simulink model "MotorFOCShared"  (R2024b)
settings: Solver=FixedStepDiscrete  StartTime=0.0  StopTime=6  FixedStep=1e-4  RelTol=1e-3
values from neighbouring files (symbols this model uses):
  CurrKi = 35.0    [motor_comparison.sldd]
  CurrKp = 0.26    [motor_comparison.sldd]
  flux = 0.016884    [motor_comparison.sldd]
  Pn = 2.0    [motor_comparison.sldd]
  spd_ki = 0.00144    [motor_comparison.sldd]
  spd_kp = 0.003389    [motor_comparison.sldd]
  Udc = 24.0    [motor_comparison.sldd]
undefined symbols (not defined in the file or in its folder): curr_d_ki, curr_d_kp, curr_q_ki, curr_q_kp, DiscIntNeverNeededParam
libraries: slpidlib x3, mcbplantlib x1, simulink x1, autolibpmsmexterior x1
settings Model: DataDictionary=motor_comparison.sldd  Creator=Administrator  LastModifiedBy=lxy
settings OptimizationCC: DefaultParameterBehavior=Inlined  UseDivisionForNetSlopeComputation=on  GainParamInheritBuiltInType=on  UseFloatMulNetSlope=on  InlineInvariantSignals=on  PassReuseOutputArgsAs=Individual arguments  ZeroExternalMemoryAtStartup=off  ZeroInternalMemoryAtStartup=off  NoFixptDivByZeroProtection=on  EfficientFloat2IntCast=on  LifeSpan=1  OptimizeBlockOrder=speed  DifferentSizesBufferReuse=on  EfficientTunableParamExpr=on
settings DebuggingCC: ParameterPrecisionLossMsg=none  ParameterTunabilityLossMsg=error  UnconnectedInputMsg=warning  UnconnectedOutputMsg=warning  UnconnectedLineMsg=warning
settings HardwareCC: ProdBitPerPointer=32  ProdBitPerSizeT=32  ProdBitPerPtrDiffT=32  ProdLargestAtomicInteger=Long  ProdLargestAtomicFloat=Double  ProdWordSize=32  ProdLongLongMode=on  ProdHWDeviceType=ARM Compatible->ARM Cortex-M
settings ModelReferenceCC: EnableRefExpFcnMdlSchedulingChecks=on  ModelReferenceNumInstancesAllowed=Single
settings SFSimCC: MATLABDynamicMemAlloc=off
settings RTWCC: Description=Embedded Coder  SystemTargetFile=ert.tlc  GenCodeOnly=on  TemplateMakefile=ert_default_tmf  GenerateReport=on  LaunchReport=on  GenerateCodeReplacementReport=on  GPUComputeCapability=3.5  DLArmComputeVersion=19.05
settings CodeAppCC: ForceParamTrailComments=on  IgnoreCustomStorageClasses=off  OperatorAnnotations=on  SimulinkDataObjDesc=on  SFDataObjDesc=on  CustomSymbolStrGlobalVar=rt$N$M  CustomSymbolStrType=$N$M  CustomSymbolStrFcn=$N$M$F  CustomSymbolStrMacro=$N$M  InsertBlockDesc=on
settings ERTTargetCC: TargetLangStandard=C99 (ISO)  GenerateSampleERTMain=on  IncludeMdlTerminateFcn=off  CombineSignalStateStructs=on  SupportComplex=off  SupportNonInlinedSFcns=on  ERTCustomFileTemplate=example_file_process.tlc  ERTFilePackagingFormat=CompactWithDataFile  DynamicArrayContainerType=coder::array

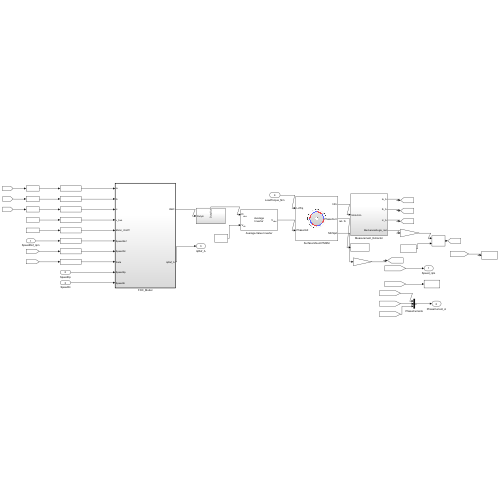
[thumbnail: Simulink's stored preview of the top-level diagram]
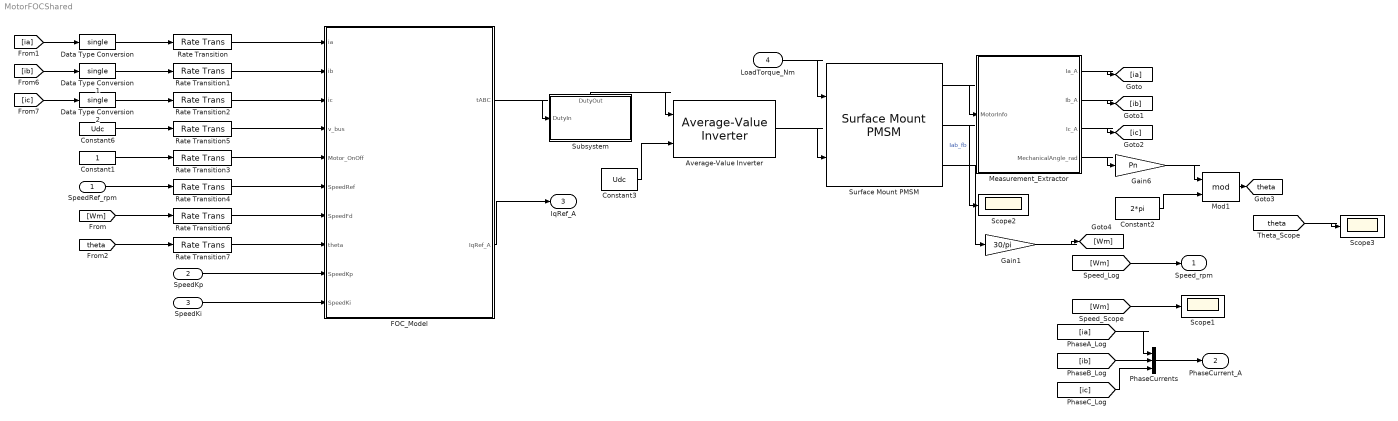
== system MotorFOCShared ==
  SpeedRef_rpm : Inport  OutDataTypeStr=single  SampleTime=1e-4
  SpeedKp : Inport  Port=2  OutDataTypeStr=single  SampleTime=1e-4
  SpeedKi : Inport  Port=3  OutDataTypeStr=single  SampleTime=1e-4
  LoadTorque_Nm : Inport  Port=4  OutDataTypeStr=double  SampleTime=1e-4
  Average-Value Inverter : mcbplantlib/Average-Value Inverter
  Constant1 : Constant  OutDataTypeStr=single
  Constant2 : Constant  Value=2*pi  OutDataTypeStr=single
  Constant3 : Constant  Value=Udc
  Constant6 : Constant  Value=Udc  OutDataTypeStr=single
  Data Type Conversion : DataTypeConversion  OutDataTypeStr=single  SaturateOnIntegerOverflow=off  RndMeth=Floor
  Data Type Conversion1 : DataTypeConversion  OutDataTypeStr=single  SaturateOnIntegerOverflow=off  RndMeth=Floor
  Data Type Conversion2 : DataTypeConversion  OutDataTypeStr=single  SaturateOnIntegerOverflow=off  RndMeth=Floor
  FOC_Model : Subsystem  TreatAsAtomicUnit=on
  Gain1 : Gain  Gain=30/pi  OutDataTypeStr=single
  Gain6 : Gain  Gain=Pn  OutDataTypeStr=single
  Measurement_Extractor : Subsystem
  Mod1 : Math  Operator=mod  OutputSignalType=real
  PhaseCurrents : Mux  Inputs=3
  Rate Transition{,1..7} (8 alike) : RateTransition
  Scope1 : Scope
  Scope2 : Scope
  Scope3 : Scope
  Subsystem : Subsystem
      settings: PortSchema="{\"entries\":[{\"content\":{\"sides\":[{\"content\":{\"connectorIds\":[\"In1\"]},\"type\":\"ConnectorPlacement.EquallySpacedRectSide\",\"uuid\":\"8ccc51de-fa2a-4900-80a3-4cdf9aa76f01\"},{\"content\":{\"connectorIds\":[],\"side\":\"RIGHT\"},\"type\":\"ConnectorPlacement.EquallySpacedRectSide\",\"uuid\":\"32c06e0d-3f1d-4948-af96-e310e54308a0\"},{\"content\":{\"connectorIds\":[\"Out1\"],\"side\":\"TOP\"},\"type\":\"ConnectorPlacement.EquallySpacedRectSide\",\"uuid\":\"a9066067-2c54-42a8-b4d7-fb86ac71b860\"}]},\"type\":\"ConnectorPlacement.EquallySpacedConnector\",\"uuid\":\"e4576975-acad-4e16-822f-2c2e7f23d7a7\"}],\"packageUris\":[\"http://schema.mathworks.com/mf0/Connector/R2020b\"],\"version\":\"1.0\"}"
  Surface Mount PMSM : autolibpmsmexterior/Surface Mount PMSM  port_config=Torque  sim_type=Discrete  Ts=1e-4  P=Pn  Rs=Rs  Ldq_=L  KConstText=Permanent flux linkage constant (lambda_pm):  lambda_pm=flux  Ke=0.0059268  Kt=0.061  mechanical=[75e-6, 8e-5, 0]  idq0=[0 0]  theta_init=4/5  omega_init=0  KConst=flux  lambda_pm_calc=flux  RefBlkName='autolibpmsmexterior/Surface Mount PMSM'  aMode=5  Ldq="[0.0017      0.0017]"
  Speed_rpm : Outport
  PhaseCurrent_A : Outport  Port=2
  IqRef_A : Outport  Port=3
  tag scope: theta=global
  wires:
  Constant3/1 -> Average-Value Inverter/2
  Subsystem/1(DutyOut) -> Average-Value Inverter/1
  Average-Value Inverter/1 -> Surface Mount PMSM/2
  Surface Mount PMSM/3 -> Gain1/1
  [ia] -> Data Type Conversion/1
  [ic] -> Data Type Conversion2/1
  [ib] -> Data Type Conversion1/1
  Data Type Conversion/1 -> Rate Transition/1
  Data Type Conversion1/1 -> Rate Transition1/1
  Data Type Conversion2/1 -> Rate Transition2/1
  Constant6/1 -> Rate Transition5/1
  Surface Mount PMSM/2 -> Scope2/1  "Iab_fb"
  Gain6/1 -> Mod1/1
  Constant2/1 -> Mod1/2
  Mod1/1 -> [theta]
  Constant1/1 -> Rate Transition3/1
  Gain1/1 -> [Wm]
  Rate Transition/1 -> FOC_Model/1(ia)
  Rate Transition1/1 -> FOC_Model/2(ib)
  Rate Transition2/1 -> FOC_Model/3(ic)
  Rate Transition5/1 -> FOC_Model/4(v_bus)
  Rate Transition3/1 -> FOC_Model/5(Motor_OnOff)
  FOC_Model/1(tABC) -> Subsystem/1(DutyIn)
  Rate Transition4/1 -> FOC_Model/6(SpeedRef)
  Rate Transition6/1 -> FOC_Model/7(SpeedFd)
  Rate Transition7/1 -> FOC_Model/8(theta)
  [theta] -> Rate Transition7/1
  [Wm] -> Rate Transition6/1
  SpeedRef_rpm/1 -> Rate Transition4/1
  LoadTorque_Nm/1 -> Surface Mount PMSM/1
  PhaseCurrents/1 -> PhaseCurrent_A/1
  SpeedKp/1 -> FOC_Model/9(SpeedKp)
  SpeedKi/1 -> FOC_Model/10(SpeedKi)
  FOC_Model/2(IqRef_A) -> IqRef_A/1
  [ia] -> PhaseCurrents/1
  [ib] -> PhaseCurrents/2
  [ic] -> PhaseCurrents/3
  [Wm] -> Speed_rpm/1
  [Wm] -> Scope1/1
  [theta] -> Scope3/1
  Surface Mount PMSM/1 -> Measurement_Extractor/1(MotorInfo)
  Measurement_Extractor/1(Ia_A) -> [ia]
  Measurement_Extractor/2(Ib_A) -> [ib]
  Measurement_Extractor/3(Ic_A) -> [ic]
  Measurement_Extractor/4(MechanicalAngle_rad) -> Gain6/1

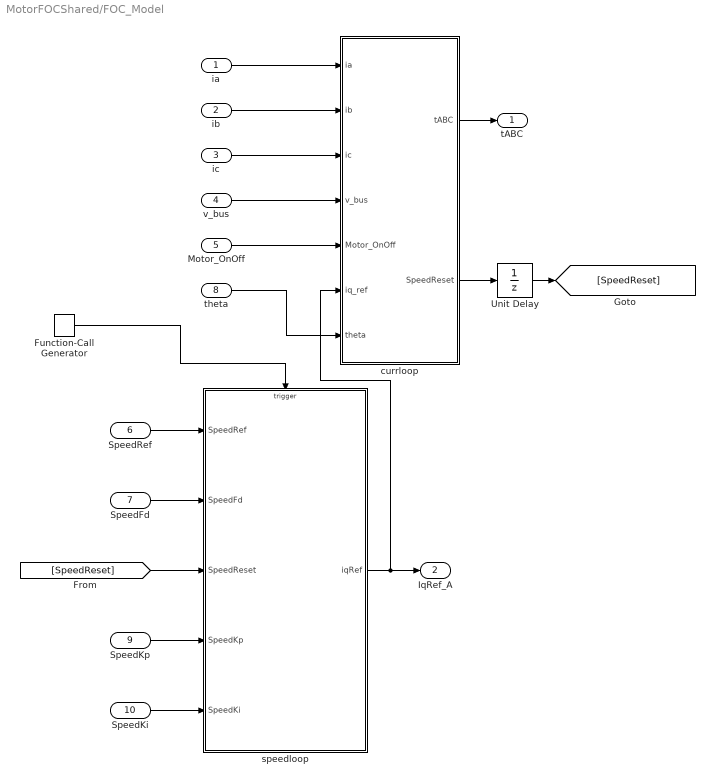
== system MotorFOCShared/FOC_Model ==
  ia : Inport
  ib : Inport  Port=2
  ic : Inport  Port=3
  v_bus : Inport  Port=4
  Motor_OnOff : Inport  Port=5
  SpeedRef : Inport  Port=6
  SpeedFd : Inport  Port=7
  theta : Inport  Port=8
  SpeedKp : Inport  Port=9  OutDataTypeStr=single
  SpeedKi : Inport  Port=10  OutDataTypeStr=single
  Function-Call Generator : simulink/Ports & Subsystems/Function-Call Generator  sample_time=1e-3  numberOfIterations=1  DisallowWideOutput=off
  Unit Delay : UnitDelay  SampleTime=-1  HasFrameUpgradeWarning=on
  currloop : Subsystem  TreatAsAtomicUnit=on
  speedloop : Subsystem
  tABC : Outport
  IqRef_A : Outport  Port=2
  wires:
  SpeedKi/1 -> speedloop/5(SpeedKi)
  SpeedKp/1 -> speedloop/4(SpeedKp)
  currloop/1(tABC) -> tABC/1
  [SpeedReset] -> speedloop/3(SpeedReset)
  theta/1 -> currloop/7(theta)
  Function-Call Generator/1 -> speedloop/Trigger
  SpeedRef/1 -> speedloop/1(SpeedRef)
  ib/1 -> currloop/2(ib)
  Motor_OnOff/1 -> currloop/5(Motor_OnOff)
  ia/1 -> currloop/1(ia)
  ic/1 -> currloop/3(ic)
  SpeedFd/1 -> speedloop/2(SpeedFd)
  v_bus/1 -> currloop/4(v_bus)
  speedloop/1(iqRef) -> IqRef_A/1, currloop/6(iq_ref)
  currloop/2(SpeedReset) -> Unit Delay/1
  Unit Delay/1 -> [SpeedReset]

== system MotorFOCShared/Measurement_Extractor ==
  MotorInfo : Inport
  Phase_And_Position : BusSelector  OutputSignals=IaStator,IbStator,IcStator,MtrPos
  Ia_A : Outport
  Ib_A : Outport  Port=2
  Ic_A : Outport  Port=3
  MechanicalAngle_rad : Outport  Port=4
  wires:
  Phase_And_Position/4 -> MechanicalAngle_rad/1  "<MtrPos>"
  Phase_And_Position/2 -> Ib_A/1  "<IbStator>"
  MotorInfo/1 -> Phase_And_Position/1
  Phase_And_Position/3 -> Ic_A/1  "<IcStator>"
  Phase_And_Position/1 -> Ia_A/1  "<IaStator>"

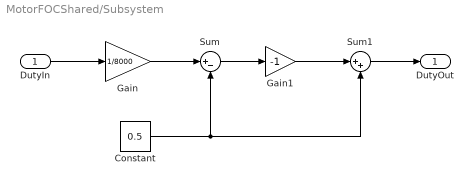
== system MotorFOCShared/Subsystem ==
  DutyIn : Inport
  Constant : Constant  Value=0.5  SampleTime=-1
  Gain : Gain  Gain=1/8000  ParamDataTypeStr=single
  Gain1 : Gain  Gain=-1
  Sum : Sum  Inputs=|+-
  Sum1 : Sum  Inputs=|++
  DutyOut : Outport
  wires:
  Sum/1 -> Gain1/1
  Constant/1 -> Sum1/2, Sum/2
  DutyIn/1 -> Gain/1
  Gain1/1 -> Sum1/1
  Sum1/1 -> DutyOut/1
  Gain/1 -> Sum/1

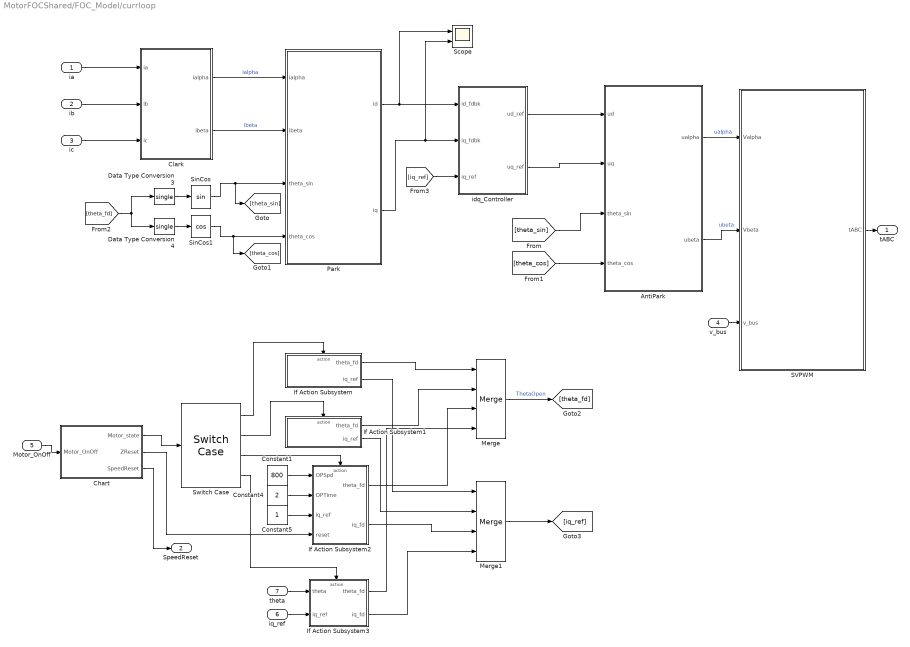
== system MotorFOCShared/FOC_Model/currloop ==
  ia : Inport
  ib : Inport  Port=2
  ic : Inport  Port=3
  v_bus : Inport  Port=4
  Motor_OnOff : Inport  Port=5
  iq_ref : Inport  Port=6
  theta : Inport  Port=7
  AntiPark : Subsystem
  Chart : Stateflow chart  TreatAsAtomicUnit=on
  Clark : Subsystem
  Constant1 : Constant  Value=800  OutDataTypeStr=single
  Constant4 : Constant  Value=2  OutDataTypeStr=single
  Constant5 : Constant  OutDataTypeStr=single
  Data Type Conversion3 : DataTypeConversion  OutDataTypeStr=single  SaturateOnIntegerOverflow=off  RndMeth=Floor
  Data Type Conversion4 : DataTypeConversion  OutDataTypeStr=single  SaturateOnIntegerOverflow=off  RndMeth=Floor
  If Action Subsystem : Subsystem  TreatAsAtomicUnit=on
  If Action Subsystem1 : Subsystem  TreatAsAtomicUnit=on
  If Action Subsystem2 : Subsystem  TreatAsAtomicUnit=on
  If Action Subsystem3 : Subsystem  TreatAsAtomicUnit=on
  Merge : Merge  Inputs=4
  Merge1 : Merge  Inputs=4
  Park : Subsystem
  SVPWM : Subsystem  TreatAsAtomicUnit=on
  Scope : Scope  NumInputPorts=2
  SinCos : Trigonometry
  SinCos1 : Trigonometry  Operator=cos
  Switch Case : SwitchCase  CaseConditions={1,2,3,4}  ShowDefaultCase=off
  idq_Controller : Subsystem
  tABC : Outport
  SpeedReset : Outport  Port=2
  wires:
  Data Type Conversion4/1 -> SinCos1/1
  Data Type Conversion3/1 -> SinCos/1
  AntiPark/2(ubeta) -> SVPWM/2(Vbeta)  "ubeta"
  AntiPark/1(ualpha) -> SVPWM/1(Valpha)  "ualpha"
  [theta_cos] -> AntiPark/4(theta_cos)
  [theta_sin] -> AntiPark/3(theta_sin)
  SinCos/1 -> Park/3(theta_sin), [theta_sin]
  [theta_fd] -> Data Type Conversion3/1, Data Type Conversion4/1
  SinCos1/1 -> Park/4(theta_cos), [theta_cos]
  v_bus/1 -> SVPWM/3(v_bus)
  SVPWM/1(tABC) -> tABC/1
  ib/1 -> Clark/2(ib)
  ia/1 -> Clark/1(ia)
  ic/1 -> Clark/3(ic)
  Clark/1(ialpha) -> Park/1(ialpha)  "ialpha"
  Clark/2(ibeta) -> Park/2(ibeta)  "ibeta"
  idq_Controller/1(ud_ref) -> AntiPark/1(ud)
  idq_Controller/2(uq_ref) -> AntiPark/2(uq)
  Park/1(id) -> Scope/1, idq_Controller/1(id_fdbk)
  Park/2(iq) -> Scope/2, idq_Controller/2(iq_fdbk)
  [iq_ref] -> idq_Controller/3(iq_ref)
  Constant1/1 -> If Action Subsystem2/1(OPSpd)
  iq_ref/1 -> If Action Subsystem3/2(iq_ref)
  Switch Case/2 -> If Action Subsystem1/Action
  Chart/1(Motor_state) -> Switch Case/1
  theta/1 -> If Action Subsystem3/1(theta)
  Switch Case/4 -> If Action Subsystem3/Action
  Constant4/1 -> If Action Subsystem2/2(OPTime)
  Constant5/1 -> If Action Subsystem2/3(iq_ref)
  Switch Case/1 -> If Action Subsystem/Action
  Switch Case/3 -> If Action Subsystem2/Action
  If Action Subsystem/1(theta_fd) -> Merge/1
  If Action Subsystem1/1(theta_fd) -> Merge/2
  If Action Subsystem2/1(theta_fd) -> Merge/3
  If Action Subsystem3/1(theta_fd) -> Merge/4
  If Action Subsystem/2(iq_ref) -> Merge1/1
  If Action Subsystem1/2(iq_ref) -> Merge1/2
  If Action Subsystem2/2(iq_fd) -> Merge1/3
  If Action Subsystem3/2(iq_fd) -> Merge1/4
  Merge/1 -> [theta_fd]  "ThetaOpen"
  Merge1/1 -> [iq_ref]
  Motor_OnOff/1 -> Chart/1(Motor_OnOff)
  Chart/2(ZReset) -> If Action Subsystem2/4(reset)
  Chart/3(SpeedReset) -> SpeedReset/1

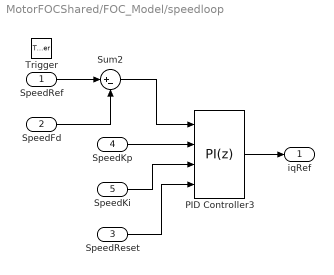
== system MotorFOCShared/FOC_Model/speedloop ==
  SpeedRef : Inport
  SpeedFd : Inport  Port=2
  SpeedReset : Inport  Port=3
  SpeedKp : Inport  Port=4  OutDataTypeStr=single
  SpeedKi : Inport  Port=5  OutDataTypeStr=single
  Trigger : TriggerPort  TriggerType=function-call  VariantControl=(inherit)  PortDimensions=1
  PID Controller3 : slpidlib/PID Controller  Controller=PI  Form=Parallel  TimeDomain=Discrete-time  UseExternalTs=off  SampleTime=-1  IntegratorMethod=Forward Euler  FilterMethod=Forward Euler  ControllerParametersSource=external  P=spd_kp  I=spd_ki  UseKiTs=off  D=0  UseExternalDerivativeSource=off  N=100  UseFilter=on  TunerSelectOption=Transfer Function Based (PID Tuner App)  InitialConditionSource=internal  InitialConditionForIntegrator=0  InitialConditionForFilter=0  DifferentiatorICPrevScaledInput=0  ExternalReset=rising  TrackingMode=off  Kt=1  LimitOutput=on  SatLimitsSource=internal  UpperSaturationLimit=3  LowerSaturationLimit=-3  LinearizeAsGain=on  AntiWindupMode=clamping  Kb=0.013  LimitIntegrator=off  UpperIntegratorSaturationLimit=inf  LowerIntegratorSaturationLimit=-inf  PGainOutDataTypeStr=single  PProdOutDataTypeStr=single  POutMin=[]  POutMax=[]  IGainOutDataTypeStr=single  IProdOutDataTypeStr=single  IOutMin=[]  IOutMax=[]  DOutMin=[]  DOutMax=[]  NOutMin=[]  NOutMax=[]  SumOutDataTypeStr=single  SumOutMin=[]  SumOutMax=[]  SaturationOutDataTypeStr=single  SaturationOutMin=[]  SaturationOutMax=[]  PParamMin=[]  PParamMax=[]  IParamMin=[]  IParamMax=[]  DParamMin=[]  DParamMax=[]  NParamMin=[]  NParamMax=[]  KbParamMin=[]  KbParamMax=[]  KtParamMin=[]  KtParamMax=[]  KbOutMin=[]  KbOutMax=[]  KtOutMin=[]  KtOutMax=[]  IntegratorOutMin=[]  IntegratorOutMax=[]  FilterOutMin=[]  FilterOutMax=[]  SumI1OutMin=[]  SumI1OutMax=[]  SumI2OutMin=[]  SumI2OutMax=[]  SumI3OutMin=[]  SumI3OutMax=[]  SumI4OutMin=[]  SumI4OutMax=[]  SumDOutMin=[]  SumDOutMax=[]  DifferentiatorOutMin=[]  DifferentiatorOutMax=[]  FilterDiffOutCoefMin=[]  FilterDiffOutCoefMax=[]  ReciprocalOutMin=[]  ReciprocalOutMax=[]  SumDenOutMin=[]  SumDenOutMax=[]  SumNumOutMin=[]  SumNumOutMax=[]  DivideOutMin=[]  DivideOutMax=[]  UdiffTsProdOutMin=[]  UdiffTsProdOutMax=[]  NTsProdOutMin=[]  NTsProdOutMax=[]  UintegralTsProdOutMin=[]  UintegralTsProdOutMax=[]  UngainTsProdOutMin=[]  UngainTsProdOutMax=[]  ClampingZeroOutDataTypeStr=Inherit: Inherit via back propagation  ClampingZeroOutMin=[]  ClampingZeroOutMax=[]  FilterDenConstantOutDataTypeStr=Inherit: Inherit via back propagation  FilterDenConstantOutMin=[]  FilterDenConstantOutMax=[]  PCopyOutDataTypeStr=Inherit: Inherit via back propagation  PCopyOutMin=[]  PCopyOutMax=[]  NCopyOutDataTypeStr=Inherit: Inherit via back propagation  NCopyOutMin=[]  NCopyOutMax=[]  IntegratorContinuousStateAttributes=''  IntegratorStateMustResolveToSignalObject=off  IntegratorRTWStateStorageClass=Auto  FilterContinuousStateAttributes=''  FilterStateMustResolveToSignalObject=off  FilterRTWStateStorageClass=Auto  ParallelPVariant=ExternalParameters  IdealPVariant=Disabled  IVariant=ExternalParameters  DVariant=Disabled  IntegratorVariant=Discrete  SatVariant=Enabled  AWVariant=DiscClampingParallel  PCopyVariant=Disabled  TRVariant=Disabled  FdbkBlocksVariant=Forward  IdealPFdbkVariant=Disabled  SatFdbkVariant=Disabled  DerivativeFilterVariant=Disabled  NVariant=Disabled  NCopyVariant=Disabled_SignalSpec  FilterICVariant=Disabled  IntegratorICVariant=InternalICs  ExternalResetVariant=ExternalReset  TRSumVariant=Passthrough  SumFdbkVariant=Disabled  SumVariant=Sum_PI  TsampFilterVariant=InternalTs  TsampNgainVariant=Passthrough  TsampIntegralVariant=Disabled_SignalSpec  ExternalSaturationOutDataTypeStr=single  DerivativeSourceVariant=Disabled  PreIntVariant=InternalPreInt
  Sum2 : Sum  Inputs=|+-  OutDataTypeStr=single  AccumDataTypeStr=single
  iqRef : Outport
  wires:
  SpeedReset/1 -> PID Controller3/4
  SpeedKi/1 -> PID Controller3/3
  SpeedKp/1 -> PID Controller3/2
  SpeedFd/1 -> Sum2/2
  SpeedRef/1 -> Sum2/1
  PID Controller3/1 -> iqRef/1
  Sum2/1 -> PID Controller3/1

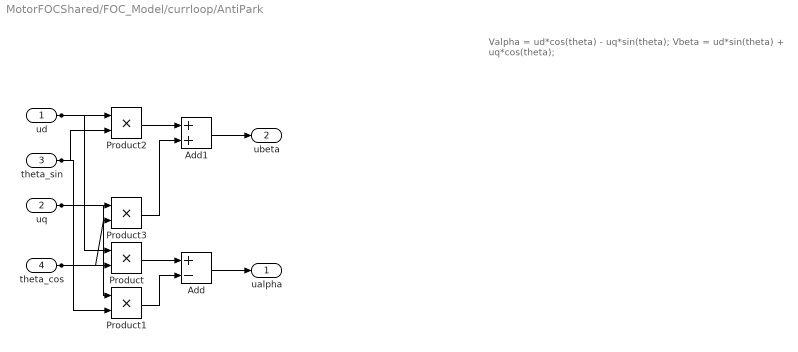
== system MotorFOCShared/FOC_Model/currloop/AntiPark ==
  note: Valpha = ud*cos(theta) - uq*sin(theta);
      | Vbeta = ud*sin(theta) + uq*cos(theta);
  ud : Inport
  uq : Inport  Port=2
  theta_sin : Inport  Port=3
  theta_cos : Inport  Port=4
  Add : Sum  Inputs=+-
  Add1 : Sum
  Product{,1..3} (4 alike) : Product
  ualpha : Outport  OutDataTypeStr=single
  ubeta : Outport  Port=2  OutDataTypeStr=single
  wires:
  ud/1 -> Product/1, Product2/1
  theta_sin/1 -> Product1/2, Product2/2
  Product/1 -> Add/1
  Product2/1 -> Add1/1
  Add/1 -> ualpha/1
  uq/1 -> Product1/1, Product3/1
  Product3/1 -> Add1/2
  theta_cos/1 -> Product3/2, Product/2
  Product1/1 -> Add/2
  Add1/1 -> ubeta/1

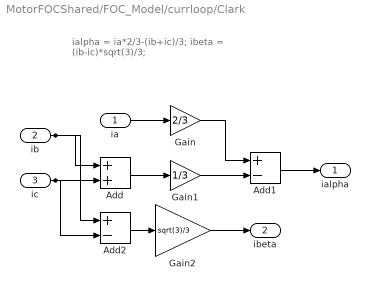
== system MotorFOCShared/FOC_Model/currloop/Clark ==
  note: ialpha = ia*2/3-(ib+ic)/3;
      | ibeta = (ib-ic)*sqrt(3)/3;
  ia : Inport  OutDataTypeStr=single
  ib : Inport  Port=2  OutDataTypeStr=single
  ic : Inport  Port=3  OutDataTypeStr=single
  Add : Sum  OutDataTypeStr=single  AccumDataTypeStr=single
  Add1 : Sum  Inputs=+-  OutDataTypeStr=single  AccumDataTypeStr=single
  Add2 : Sum  Inputs=+-  OutDataTypeStr=single  AccumDataTypeStr=single
  Gain : Gain  Gain=2/3  ParamDataTypeStr=single
  Gain1 : Gain  Gain=1/3  ParamDataTypeStr=single
  Gain2 : Gain  Gain=sqrt(3)/3  ParamDataTypeStr=single
  ialpha : Outport  OutDataTypeStr=single
  ibeta : Outport  Port=2  OutDataTypeStr=single
  wires:
  ib/1 -> Add/1, Add2/1
  Gain/1 -> Add1/1
  ic/1 -> Add/2, Add2/2
  Gain2/1 -> ibeta/1
  Gain1/1 -> Add1/2
  ia/1 -> Gain/1
  Add2/1 -> Gain2/1
  Add/1 -> Gain1/1
  Add1/1 -> ialpha/1

== system MotorFOCShared/FOC_Model/currloop/If Action Subsystem ==
  Action Port : ActionPort  ActionPortLabel=case [ 1 ]:
  Constant : Constant  Value=0  OutDataTypeStr=single
  Constant1 : Constant  Value=0  OutDataTypeStr=single
  theta_fd : Outport
  iq_ref : Outport  Port=2
  wires:
  Constant1/1 -> iq_ref/1
  Constant/1 -> theta_fd/1

== system MotorFOCShared/FOC_Model/currloop/If Action Subsystem1 ==
  Action Port : ActionPort  ActionPortLabel=case [ 2 ]:
  Constant : Constant  Value=0  OutDataTypeStr=single
  Constant1 : Constant  OutDataTypeStr=single
  theta_fd : Outport
  iq_ref : Outport  Port=2
  wires:
  Constant1/1 -> iq_ref/1
  Constant/1 -> theta_fd/1

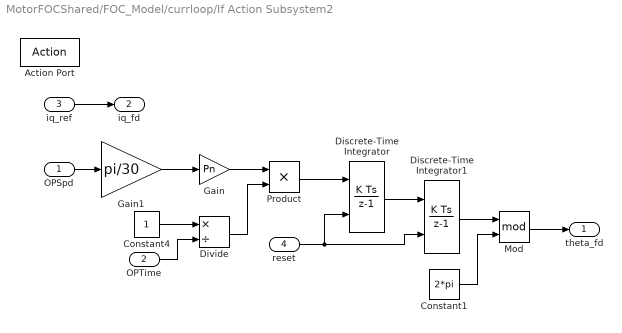
== system MotorFOCShared/FOC_Model/currloop/If Action Subsystem2 ==
  OPSpd : Inport  OutDataTypeStr=single  PortDimensions=1
  OPTime : Inport  Port=2  OutDataTypeStr=single  PortDimensions=1
  iq_ref : Inport  Port=3
  reset : Inport  Port=4
  Action Port : ActionPort  ActionPortLabel=case [ 3 ]:
  Constant1 : Constant  Value=2*pi  OutDataTypeStr=single
  Constant4 : Constant  OutDataTypeStr=single
  Discrete-Time Integrator : DiscreteIntegrator  ExternalReset=rising  SampleTime=-1  ICPrevOutput=DiscIntNeverNeededParam  ICPrevScaledInput=DiscIntNeverNeededParam
  Discrete-Time Integrator1 : DiscreteIntegrator  ExternalReset=rising  SampleTime=-1  ICPrevOutput=DiscIntNeverNeededParam  ICPrevScaledInput=DiscIntNeverNeededParam
  Divide : Product  Inputs=*/  OutDataTypeStr=single
  Gain : Gain  Gain=Pn
  Gain1 : Gain  Gain=pi/30  OutDataTypeStr=single
  Mod : Math  Operator=mod
  Product : Product  OutDataTypeStr=single
  theta_fd : Outport
  iq_fd : Outport  Port=2
  wires:
  Gain/1 -> Product/1
  Discrete-Time Integrator1/1 -> Mod/1
  OPTime/1 -> Divide/2
  Mod/1 -> theta_fd/1
  OPSpd/1 -> Gain1/1
  iq_ref/1 -> iq_fd/1
  Product/1 -> Discrete-Time Integrator/1
  Divide/1 -> Product/2
  Constant4/1 -> Divide/1
  Gain1/1 -> Gain/1
  reset/1 -> Discrete-Time Integrator1/2, Discrete-Time Integrator/2
  Discrete-Time Integrator/1 -> Discrete-Time Integrator1/1
  Constant1/1 -> Mod/2

== system MotorFOCShared/FOC_Model/currloop/If Action Subsystem3 ==
  theta : Inport  OutDataTypeStr=single  PortDimensions=1
  iq_ref : Inport  Port=2
  Action Port : ActionPort  ActionPortLabel=case [ 4 ]:
  theta_fd : Outport
  iq_fd : Outport  Port=2
  wires:
  iq_ref/1 -> iq_fd/1
  theta/1 -> theta_fd/1

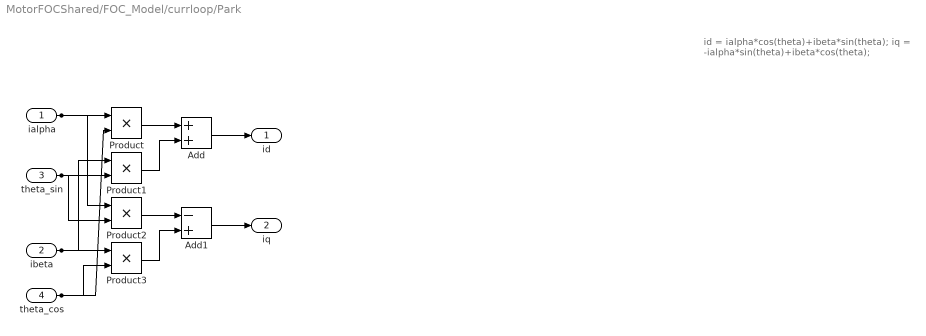
== system MotorFOCShared/FOC_Model/currloop/Park ==
  note: id = ialpha*cos(theta)+ibeta*sin(theta);
      | iq = -ialpha*sin(theta)+ibeta*cos(theta);
  ialpha : Inport  OutDataTypeStr=single
  ibeta : Inport  Port=2  OutDataTypeStr=single
  theta_sin : Inport  Port=3  OutDataTypeStr=single
  theta_cos : Inport  Port=4  OutDataTypeStr=single
  Add : Sum  OutDataTypeStr=single  AccumDataTypeStr=single
  Add1 : Sum  Inputs=-+  OutDataTypeStr=single  AccumDataTypeStr=single
  Product{,1..3} (4 alike) : Product  OutDataTypeStr=single
  id : Outport  OutDataTypeStr=single
  iq : Outport  Port=2  OutDataTypeStr=single
  wires:
  Product3/1 -> Add1/2
  Product1/1 -> Add/2
  ialpha/1 -> Product/1, Product2/1
  theta_sin/1 -> Product1/2, Product2/2
  ibeta/1 -> Product1/1, Product3/1
  Add/1 -> id/1
  theta_cos/1 -> Product/2, Product3/2
  Product2/1 -> Add1/1
  Product/1 -> Add/1
  Add1/1 -> iq/1

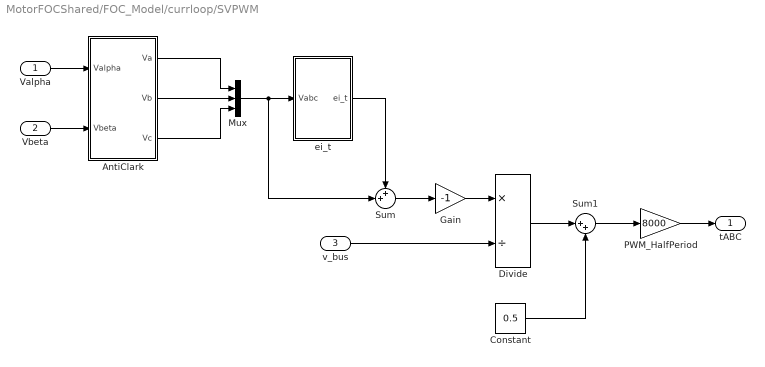
== system MotorFOCShared/FOC_Model/currloop/SVPWM ==
  Valpha : Inport  OutDataTypeStr=single
  Vbeta : Inport  Port=2  OutDataTypeStr=single
  v_bus : Inport  Port=3  OutDataTypeStr=single
  AntiClark : Subsystem
  Constant : Constant  Value=0.5  OutDataTypeStr=single
  Divide : Product  Inputs=*/  OutDataTypeStr=single
  Gain : Gain  Gain=-1  OutDataTypeStr=single
  Mux : Mux  Inputs=3
  PWM_HalfPeriod : Gain  Gain=8000  OutDataTypeStr=single
  Sum : Sum  Inputs=++|  OutDataTypeStr=single
  Sum1 : Sum  Inputs=|++  OutDataTypeStr=single
  ei_t : Subsystem
  tABC : Outport  OutDataTypeStr=single
  wires:
  Gain/1 -> Divide/1
  v_bus/1 -> Divide/2
  PWM_HalfPeriod/1 -> tABC/1
  Sum1/1 -> PWM_HalfPeriod/1
  Constant/1 -> Sum1/2
  Divide/1 -> Sum1/1
  Mux/1 -> ei_t/1(Vabc), Sum/2
  Sum/1 -> Gain/1
  AntiClark/3(Vc) -> Mux/3
  AntiClark/2(Vb) -> Mux/2
  AntiClark/1(Va) -> Mux/1
  ei_t/1(ei_t) -> Sum/1
  Vbeta/1 -> AntiClark/2(Vbeta)
  Valpha/1 -> AntiClark/1(Valpha)

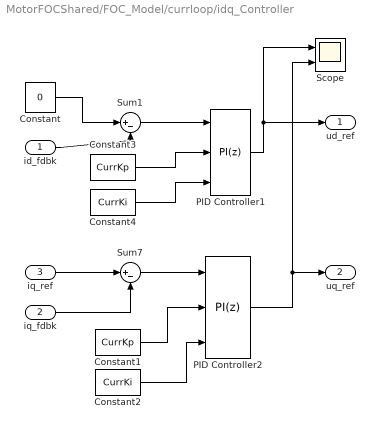
== system MotorFOCShared/FOC_Model/currloop/idq_Controller ==
  id_fdbk : Inport  OutDataTypeStr=single
  iq_fdbk : Inport  Port=2  OutDataTypeStr=single
  iq_ref : Inport  Port=3  OutDataTypeStr=single
  Constant : Constant  Value=0  OutDataTypeStr=single
  Constant1 : Constant  Value=CurrKp  OutDataTypeStr=single
  Constant2 : Constant  Value=CurrKi  OutDataTypeStr=single
  Constant3 : Constant  Value=CurrKp  OutDataTypeStr=single
  Constant4 : Constant  Value=CurrKi  OutDataTypeStr=single
  PID Controller1 : slpidlib/PID Controller  Controller=PI  Form=Parallel  TimeDomain=Discrete-time  UseExternalTs=off  SampleTime=-1  IntegratorMethod=Forward Euler  FilterMethod=Forward Euler  ControllerParametersSource=external  P=curr_d_kp  I=curr_d_ki  UseKiTs=off  D=0  UseExternalDerivativeSource=off  N=100  UseFilter=on  TunerSelectOption=Transfer Function Based (PID Tuner App)  InitialConditionSource=internal  InitialConditionForIntegrator=0  InitialConditionForFilter=0  DifferentiatorICPrevScaledInput=0  ExternalReset=none  TrackingMode=off  Kt=1  LimitOutput=on  SatLimitsSource=internal  UpperSaturationLimit=24*0.9/sqrt(3)  LowerSaturationLimit=-24*0.9/sqrt(3)  LinearizeAsGain=on  AntiWindupMode=clamping  Kb=1  LimitIntegrator=off  UpperIntegratorSaturationLimit=inf  LowerIntegratorSaturationLimit=-inf  PGainOutDataTypeStr=single  PProdOutDataTypeStr=single  POutMin=[]  POutMax=[]  IGainOutDataTypeStr=single  IProdOutDataTypeStr=single  IOutMin=[]  IOutMax=[]  DOutMin=[]  DOutMax=[]  NOutMin=[]  NOutMax=[]  SumOutDataTypeStr=single  SumOutMin=[]  SumOutMax=[]  SaturationOutDataTypeStr=single  SaturationOutMin=[]  SaturationOutMax=[]  PParamMin=[]  PParamMax=[]  IParamMin=[]  IParamMax=[]  DParamMin=[]  DParamMax=[]  NParamMin=[]  NParamMax=[]  KbParamMin=[]  KbParamMax=[]  KtParamMin=[]  KtParamMax=[]  KbOutMin=[]  KbOutMax=[]  KtOutMin=[]  KtOutMax=[]  IntegratorOutMin=[]  IntegratorOutMax=[]  FilterOutMin=[]  FilterOutMax=[]  SumI1OutMin=[]  SumI1OutMax=[]  SumI2OutMin=[]  SumI2OutMax=[]  SumI3OutMin=[]  SumI3OutMax=[]  SumI4OutMin=[]  SumI4OutMax=[]  SumDOutMin=[]  SumDOutMax=[]  DifferentiatorOutMin=[]  DifferentiatorOutMax=[]  FilterDiffOutCoefMin=[]  FilterDiffOutCoefMax=[]  ReciprocalOutMin=[]  ReciprocalOutMax=[]  SumDenOutMin=[]  SumDenOutMax=[]  SumNumOutMin=[]  SumNumOutMax=[]  DivideOutMin=[]  DivideOutMax=[]  UdiffTsProdOutMin=[]  UdiffTsProdOutMax=[]  NTsProdOutMin=[]  NTsProdOutMax=[]  UintegralTsProdOutMin=[]  UintegralTsProdOutMax=[]  UngainTsProdOutMin=[]  UngainTsProdOutMax=[]  ClampingZeroOutDataTypeStr=Inherit: Inherit via back propagation  ClampingZeroOutMin=[]  ClampingZeroOutMax=[]  FilterDenConstantOutDataTypeStr=Inherit: Inherit via back propagation  FilterDenConstantOutMin=[]  FilterDenConstantOutMax=[]  PCopyOutDataTypeStr=Inherit: Inherit via back propagation  PCopyOutMin=[]  PCopyOutMax=[]  NCopyOutDataTypeStr=Inherit: Inherit via back propagation  NCopyOutMin=[]  NCopyOutMax=[]  IntegratorContinuousStateAttributes=''  IntegratorStateMustResolveToSignalObject=off  IntegratorRTWStateStorageClass=Auto  FilterContinuousStateAttributes=''  FilterStateMustResolveToSignalObject=off  FilterRTWStateStorageClass=Auto  ParallelPVariant=ExternalParameters  IdealPVariant=Disabled  IVariant=ExternalParameters  DVariant=Disabled  IntegratorVariant=Discrete  SatVariant=Enabled  AWVariant=DiscClampingParallel  PCopyVariant=Disabled  TRVariant=Disabled  FdbkBlocksVariant=Forward  IdealPFdbkVariant=Disabled  SatFdbkVariant=Disabled  DerivativeFilterVariant=Disabled  NVariant=Disabled  NCopyVariant=Disabled_SignalSpec  FilterICVariant=Disabled  IntegratorICVariant=InternalICs  ExternalResetVariant=Disabled  TRSumVariant=Passthrough  SumFdbkVariant=Disabled  SumVariant=Sum_PI  TsampFilterVariant=InternalTs  TsampNgainVariant=Passthrough  TsampIntegralVariant=Disabled_SignalSpec  ExternalSaturationOutDataTypeStr=Inherit: Same as second input  DerivativeSourceVariant=Disabled  PreIntVariant=InternalPreInt
  PID Controller2 : slpidlib/PID Controller  Controller=PI  Form=Parallel  TimeDomain=Discrete-time  UseExternalTs=off  SampleTime=-1  IntegratorMethod=Forward Euler  FilterMethod=Forward Euler  ControllerParametersSource=external  P=curr_q_kp  I=curr_q_ki  UseKiTs=off  D=0  UseExternalDerivativeSource=off  N=100  UseFilter=on  TunerSelectOption=Transfer Function Based (PID Tuner App)  InitialConditionSource=internal  InitialConditionForIntegrator=0  InitialConditionForFilter=0  DifferentiatorICPrevScaledInput=0  ExternalReset=none  TrackingMode=off  Kt=1  LimitOutput=on  SatLimitsSource=internal  UpperSaturationLimit=24*0.9/sqrt(3)  LowerSaturationLimit=-24*0.9/sqrt(3)  LinearizeAsGain=on  AntiWindupMode=clamping  Kb=1  LimitIntegrator=off  UpperIntegratorSaturationLimit=inf  LowerIntegratorSaturationLimit=-inf  PGainOutDataTypeStr=single  PProdOutDataTypeStr=single  POutMin=[]  POutMax=[]  IGainOutDataTypeStr=single  IProdOutDataTypeStr=single  IOutMin=[]  IOutMax=[]  DOutMin=[]  DOutMax=[]  NOutMin=[]  NOutMax=[]  SumOutDataTypeStr=single  SumOutMin=[]  SumOutMax=[]  SaturationOutDataTypeStr=single  SaturationOutMin=[]  SaturationOutMax=[]  PParamMin=[]  PParamMax=[]  IParamMin=[]  IParamMax=[]  DParamMin=[]  DParamMax=[]  NParamMin=[]  NParamMax=[]  KbParamMin=[]  KbParamMax=[]  KtParamMin=[]  KtParamMax=[]  KbOutMin=[]  KbOutMax=[]  KtOutMin=[]  KtOutMax=[]  IntegratorOutMin=[]  IntegratorOutMax=[]  FilterOutMin=[]  FilterOutMax=[]  SumI1OutMin=[]  SumI1OutMax=[]  SumI2OutMin=[]  SumI2OutMax=[]  SumI3OutMin=[]  SumI3OutMax=[]  SumI4OutMin=[]  SumI4OutMax=[]  SumDOutMin=[]  SumDOutMax=[]  DifferentiatorOutMin=[]  DifferentiatorOutMax=[]  FilterDiffOutCoefMin=[]  FilterDiffOutCoefMax=[]  ReciprocalOutMin=[]  ReciprocalOutMax=[]  SumDenOutMin=[]  SumDenOutMax=[]  SumNumOutMin=[]  SumNumOutMax=[]  DivideOutMin=[]  DivideOutMax=[]  UdiffTsProdOutMin=[]  UdiffTsProdOutMax=[]  NTsProdOutMin=[]  NTsProdOutMax=[]  UintegralTsProdOutMin=[]  UintegralTsProdOutMax=[]  UngainTsProdOutMin=[]  UngainTsProdOutMax=[]  ClampingZeroOutDataTypeStr=Inherit: Inherit via back propagation  ClampingZeroOutMin=[]  ClampingZeroOutMax=[]  FilterDenConstantOutDataTypeStr=Inherit: Inherit via back propagation  FilterDenConstantOutMin=[]  FilterDenConstantOutMax=[]  PCopyOutDataTypeStr=Inherit: Inherit via back propagation  PCopyOutMin=[]  PCopyOutMax=[]  NCopyOutDataTypeStr=Inherit: Inherit via back propagation  NCopyOutMin=[]  NCopyOutMax=[]  IntegratorContinuousStateAttributes=''  IntegratorStateMustResolveToSignalObject=off  IntegratorRTWStateStorageClass=Auto  FilterContinuousStateAttributes=''  FilterStateMustResolveToSignalObject=off  FilterRTWStateStorageClass=Auto  ParallelPVariant=ExternalParameters  IdealPVariant=Disabled  IVariant=ExternalParameters  DVariant=Disabled  IntegratorVariant=Discrete  SatVariant=Enabled  AWVariant=DiscClampingParallel  PCopyVariant=Disabled  TRVariant=Disabled  FdbkBlocksVariant=Forward  IdealPFdbkVariant=Disabled  SatFdbkVariant=Disabled  DerivativeFilterVariant=Disabled  NVariant=Disabled  NCopyVariant=Disabled_SignalSpec  FilterICVariant=Disabled  IntegratorICVariant=InternalICs  ExternalResetVariant=Disabled  TRSumVariant=Passthrough  SumFdbkVariant=Disabled  SumVariant=Sum_PI  TsampFilterVariant=InternalTs  TsampNgainVariant=Passthrough  TsampIntegralVariant=Disabled_SignalSpec  ExternalSaturationOutDataTypeStr=Inherit: Same as second input  DerivativeSourceVariant=Disabled  PreIntVariant=InternalPreInt
  Scope : Scope  NumInputPorts=2
  Sum1 : Sum  Inputs=|+-  OutDataTypeStr=single  AccumDataTypeStr=single
  Sum7 : Sum  Inputs=|+-  OutDataTypeStr=single  AccumDataTypeStr=single
  ud_ref : Outport  OutDataTypeStr=single
  uq_ref : Outport  Port=2  OutDataTypeStr=single
  wires:
  id_fdbk/1 -> Sum1/2
  Constant/1 -> Sum1/1
  iq_fdbk/1 -> Sum7/2
  Sum1/1 -> PID Controller1/1
  Sum7/1 -> PID Controller2/1
  PID Controller1/1 -> Scope/1, ud_ref/1
  PID Controller2/1 -> Scope/2, uq_ref/1
  iq_ref/1 -> Sum7/1
  Constant3/1 -> PID Controller1/2
  Constant4/1 -> PID Controller1/3
  Constant1/1 -> PID Controller2/2
  Constant2/1 -> PID Controller2/3

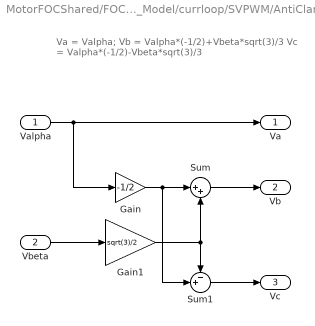
== system MotorFOCShared/FOC_Model/currloop/SVPWM/AntiClark ==
  note: Va = Valpha;
      | Vb = Valpha*(-1/2)+Vbeta*sqrt(3)/3
      | Vc = Valpha*(-1/2)-Vbeta*sqrt(3)/3
  Valpha : Inport  OutDataTypeStr=single
  Vbeta : Inport  Port=2  OutDataTypeStr=single
  Gain : Gain  Gain=-1/2  OutDataTypeStr=single
  Gain1 : Gain  Gain=sqrt(3)/2  OutDataTypeStr=single
  Sum : Sum  Inputs=|++  OutDataTypeStr=single
  Sum1 : Sum  Inputs=-+|  OutDataTypeStr=single
  Va : Outport  OutDataTypeStr=single
  Vb : Outport  Port=2  OutDataTypeStr=single
  Vc : Outport  Port=3  OutDataTypeStr=single
  wires:
  Sum1/1 -> Vc/1
  Gain1/1 -> Sum1/1, Sum/2
  Sum/1 -> Vb/1
  Gain/1 -> Sum/1, Sum1/2
  Vbeta/1 -> Gain1/1
  Valpha/1 -> Va/1, Gain/1

== system MotorFOCShared/FOC_Model/currloop/SVPWM/ei_t ==
  note: V0 = -1/2(Vmax+Vmin)
  Vabc : Inport  OutDataTypeStr=single
  Demux : Demux  Outputs=3
  Gain : Gain  Gain=-1/2  OutDataTypeStr=single
  Min : MinMax  Inputs=3  OutDataTypeStr=single
  Min1 : MinMax  Function=max  Inputs=3  OutDataTypeStr=single
  Sum : Sum  Inputs=|++  OutDataTypeStr=single
  ei_t : Outport  OutDataTypeStr=single
  wires:
  Demux/3 -> Min/3, Min1/3
  Demux/2 -> Min1/2, Min/2
  Demux/1 -> Min/1, Min1/1
  Vabc/1 -> Demux/1
  Gain/1 -> ei_t/1
  Min1/1 -> Sum/2
  Sum/1 -> Gain/1
  Min/1 -> Sum/1

== stateflow chart MotorFOCShared/FOC_Model/currloop/Chart ==
  state RunStage
    en:
    du:
    Motor_state = 4;
    SpeedReset = 1;
  state OpenStage
    en:
    ZReset = 0;
    cnt = 0;
    du:
    if cnt == 1
    ZReset = 1;
    end
    cnt = 1;
    Motor_state = 3;
    SpeedReset = 0;
  state AlignStage
    en:
    du:
    Motor_state = 2;
  state IDLE
    en:
    du:
    Motor_state = 1;
  (default) -> IDLE
  IDLE -> AlignStage : [Motor_OnOff ==1]
  AlignStage -> OpenStage [order 1] : [after(2000,tick)]
  OpenStage -> RunStage [order 2] : [after(20000,tick) ]
  AlignStage -> IDLE [order 2] : [Motor_OnOff == 0]
  RunStage -> IDLE : [Motor_OnOff ==0]
  OpenStage -> IDLE [order 1] : [Motor_OnOff ==0]
  data: Motor_OnOff input; Motor_state output; cnt local; ZReset output; SpeedReset output
